simulink library "fmCopterAltHoldIndi_lib"  (R2018b)
settings: Solver=VariableStepAuto  StartTime=0.0  StopTime=10.0  RelTol=1e-3
undefined symbols (not defined in the file or in its folder): fm_alt_hold
libraries: filters_lib x5, indi_lib x1, cntrlAttiRedIndi_lib x1, cntrlAltIndi_lib x1
settings Model: Creator=Ybeyer  LastModifiedBy=yannic
settings SFSimCC: SimUseLocalCustomCode=off
settings RTWCC: RTWUseLocalCustomCode=off
settings CodeAppCC: StateflowObjectComments=on

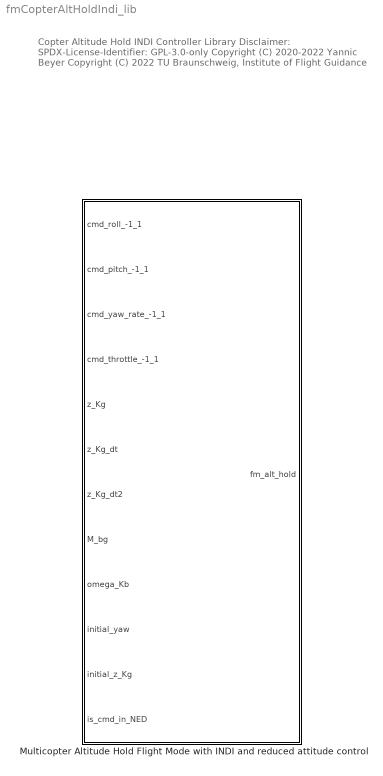
== system fmCopterAltHoldIndi_lib ==
  note: Copter Altitude Hold INDI Controller Library
      |
      | Disclaimer:
      | SPDX-License-Identifier: GPL-3.0-only
      |
      | Copyright (C) 2020-2022 Yannic Beyer
      | Copyright (C) 2022 TU Braunschweig, Institute of Flight Guidance
  Multicopter Altitude Hold Flight Mode with INDI and reduced attitude control : Subsystem  mask{fm=fm_alt_hold}
      mask prompts: fm "Multicopter Altitude Hold Flight Mode (INDI) struct, see fmCopterAltHoldIndi_params_default"
      mask DialogControl DescGroupVar Prompt: Multicopter Attitude Flight Mode with INDI and reduced attitude control
      mask DialogControl DescTextVar Prompt: Controller is basically implemented according to [1]
      mask DialogControl Control2 Prompt: [1] Sun, S., Baert, M., Van Schijndel, B. S., & De Visser, C. (2020, May). Upset Recovery Control for Quadrotors Subjected to a Complete Rotor Failure from Large Initial Disturbances. In 2020 IEEE International Conference on Robotics and Automation (ICRA) (pp. 4273-4279). IEEE.

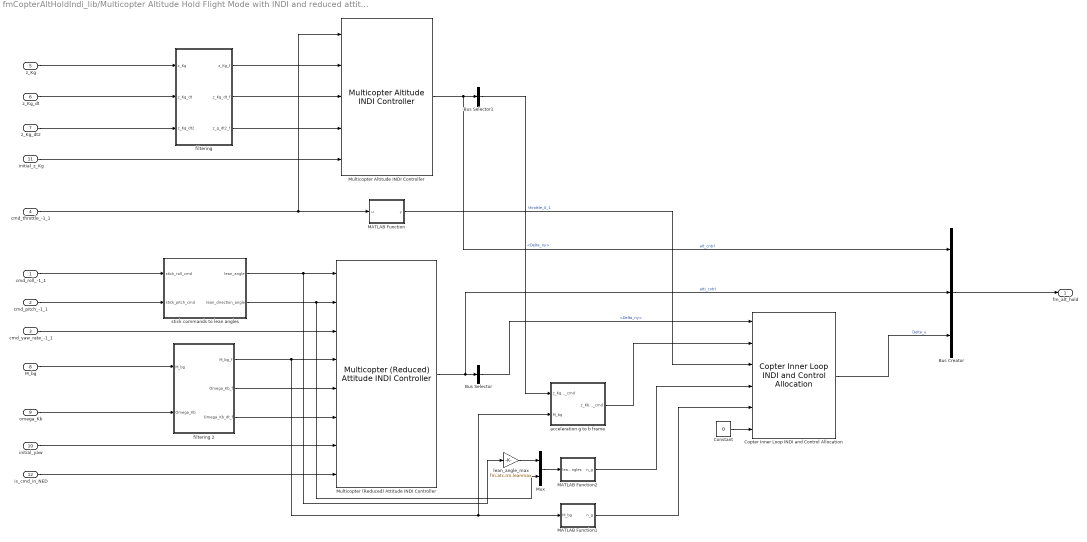
== system fmCopterAltHoldIndi_lib/Multicopter Altitude Hold Flight Mode with INDI and reduced attitude control ==
  cmd_roll_-1_1 : Inport  SampleTime=fm.ts
  cmd_pitch_-1_1 : Inport  Port=2  SampleTime=fm.ts
  cmd_yaw_rate_-1_1 : Inport  Port=3  SampleTime=fm.ts
  cmd_throttle_-1_1 : Inport  Port=4  SampleTime=fm.ts
  z_Kg : Inport  Port=5  SampleTime=fm.ts
  z_Kg_dt : Inport  Port=6  SampleTime=fm.ts
  z_Kg_dt2 : Inport  Port=7  SampleTime=fm.ts
  M_bg : Inport  Port=8  SampleTime=fm.ts
  omega_Kb : Inport  Port=9  SampleTime=fm.ts
  initial_yaw : Inport  Port=10  SampleTime=fm.ts
  initial_z_Kg : Inport  Port=11  SampleTime=fm.ts
  is_cmd_in_NED : Inport  Port=12  SampleTime=fm.ts
  Bus Creator : BusCreator  Inputs=3
  Bus Selector : BusSelector  OutputSignals=pseudo_control.Delta_ny
  Bus Selector1 : BusSelector  OutputSignals=pseudo_control.Delta_ny
  Constant : Constant  Value=0
  Copter Inner Loop INDI and Control Allocation : indi_lib/Copter Inner Loop INDI and Control Allocation  cep=fm.cep  ceb=fm.ceb  ca=fm.ca  mtc=fm.mtc  sflt=fm.sflt  ts=fm.ts
      settings: SourceProductName=LADAC
  MATLAB Function : MATLAB Function  TreatAsAtomicUnit=on
  MATLAB Function1 : MATLAB Function  TreatAsAtomicUnit=on
  MATLAB Function2 : MATLAB Function  TreatAsAtomicUnit=on
  Multicopter (Reduced) Attitude INDI Controller : cntrlAttiRedIndi_lib/Multicopter (Reduced) Attitude INDI Controller  atc=fm.atc  T=fm.mtc + 2./fm.sflt.omega
      settings: SourceProductName=LADAC
  Multicopter Altitude INDI Controller : cntrlAltIndi_lib/Multicopter Altitude INDI Controller  psc=fm.psc
      settings: SourceProductName=LADAC
  Mux : Mux  Inputs=2
  acceleration g to b frame : Subsystem
  filtering : Subsystem
  filtering 2 : Subsystem
  lean_angle_max : Gain  Gain=fm.atc.rm.leanmax
  stick commands to lean angles : MATLAB Function  TreatAsAtomicUnit=on
  fm_alt_hold : Outport  SampleTime=fm.ts
  wires:
  is_cmd_in_NED/1 -> Multicopter (Reduced) Attitude INDI Controller/8
  Multicopter Altitude INDI Controller/1 -> Bus Creator/1, Bus Selector1/1  "alt_cntrl"
  cmd_yaw_rate_-1_1/1 -> Multicopter (Reduced) Attitude INDI Controller/3
  stick commands to lean angles/2(lean_direction_angle) -> Mux/2, Multicopter (Reduced) Attitude INDI Controller/2
  Bus Selector1/1 -> acceleration g to b frame/1(z_Kg_dt2_cmd)  "<Delta_ny>"
  MATLAB Function/1(y) -> Copter Inner Loop INDI and Control Allocation/3  "throttle_0_1"
  cmd_throttle_-1_1/1 -> MATLAB Function/1(u), Multicopter Altitude INDI Controller/1
  Multicopter (Reduced) Attitude INDI Controller/1 -> Bus Creator/2, Bus Selector/1  "atti_cntrl"
  initial_yaw/1 -> Multicopter (Reduced) Attitude INDI Controller/7
  stick commands to lean angles/1(lean_angle) -> lean_angle_max/1, Multicopter (Reduced) Attitude INDI Controller/1
  Bus Selector/1 -> Copter Inner Loop INDI and Control Allocation/1  "<Delta_ny>"
  filtering 2/3(Omega_Kb_dt_f) -> Multicopter (Reduced) Attitude INDI Controller/6
  filtering 2/2(Omega_Kb_f) -> Multicopter (Reduced) Attitude INDI Controller/5
  filtering/1(z_Kg_f) -> Multicopter Altitude INDI Controller/2
  filtering/2(z_Kg_dt_f) -> Multicopter Altitude INDI Controller/3
  filtering/3(z_g_dt2_f) -> Multicopter Altitude INDI Controller/4
  initial_z_Kg/1 -> Multicopter Altitude INDI Controller/5
  Bus Creator/1 -> fm_alt_hold/1
  cmd_roll_-1_1/1 -> stick commands to lean angles/1(stick_roll_cmd)
  cmd_pitch_-1_1/1 -> stick commands to lean angles/2(stick_pitch_cmd)
  filtering 2/1(M_bg_f) -> Multicopter (Reduced) Attitude INDI Controller/4, acceleration g to b frame/2(M_bg), MATLAB Function1/1(M_bg)
  acceleration g to b frame/1(z_Kb_dt2_cmd) -> Copter Inner Loop INDI and Control Allocation/2
  Copter Inner Loop INDI and Control Allocation/1 -> Bus Creator/3  "Delta_u"
  z_Kg/1 -> filtering/1(z_Kg)
  z_Kg_dt/1 -> filtering/2(z_Kg_dt)
  z_Kg_dt2/1 -> filtering/3(z_Kg_dt2)
  M_bg/1 -> filtering 2/1(M_bg)
  omega_Kb/1 -> filtering 2/2(Omega_Kb)
  MATLAB Function1/1(n_g) -> Copter Inner Loop INDI and Control Allocation/5
  MATLAB Function2/1(n_g) -> Copter Inner Loop INDI and Control Allocation/4
  lean_angle_max/1 -> Mux/1
  Mux/1 -> MATLAB Function2/1(leanAngles)
  Constant/1 -> Copter Inner Loop INDI and Control Allocation/6

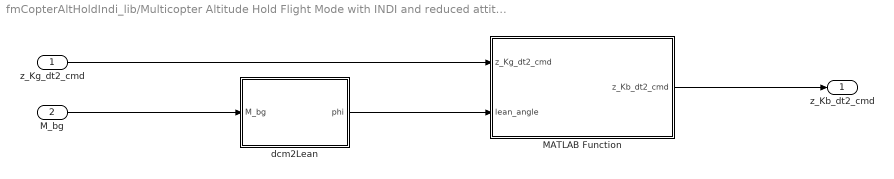
== system fmCopterAltHoldIndi_lib/Multicopter Altitude Hold Flight Mode with INDI and reduced attitude control/acceleration g to b frame ==
  z_Kg_dt2_cmd : Inport
  M_bg : Inport  Port=2
  MATLAB Function : MATLAB Function  TreatAsAtomicUnit=on
  dcm2Lean : MATLAB Function  TreatAsAtomicUnit=on
  z_Kb_dt2_cmd : Outport
  wires:
  z_Kg_dt2_cmd/1 -> MATLAB Function/1(z_Kg_dt2_cmd)
  MATLAB Function/1(z_Kb_dt2_cmd) -> z_Kb_dt2_cmd/1
  M_bg/1 -> dcm2Lean/1(M_bg)
  dcm2Lean/1(phi) -> MATLAB Function/2(lean_angle)

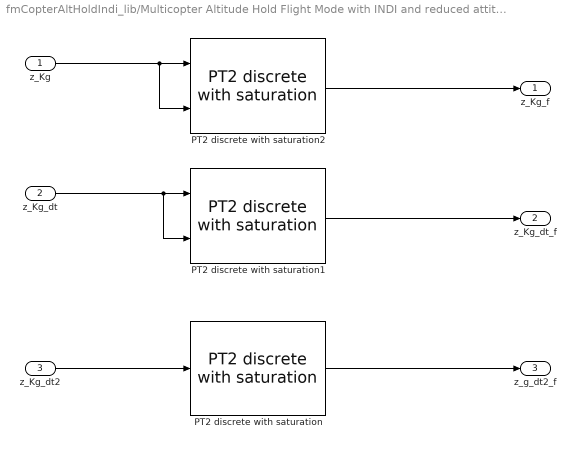
== system fmCopterAltHoldIndi_lib/Multicopter Altitude Hold Flight Mode with INDI and reduced attitude control/filtering ==
  z_Kg : Inport
  z_Kg_dt : Inport  Port=2
  z_Kg_dt2 : Inport  Port=3
  PT2 discrete with saturation : filters_lib/PT2 discrete with saturation  param_src=internal  omega=fm.sflt.omega  d=fm.sflt.D  x_dt2_max=inf  x_dt2_min=-inf  x_dt_max=inf  x_dt_min=-inf  x_max=inf  x_min=-inf  y_0_src=internal  x_init=0  y_dt_0_src=internal  x_dt_init=0  is_y_dt_checked=off  is_y_dt2_checked=off
      settings: SourceProductName=LADAC
  PT2 discrete with saturation1 : filters_lib/PT2 discrete with saturation  param_src=internal  omega=fm.sflt.omega  d=fm.sflt.D  x_dt2_max=inf  x_dt2_min=-inf  x_dt_max=inf  x_dt_min=-inf  x_max=inf  x_min=-inf  y_0_src=external  x_init=0  y_dt_0_src=internal  x_dt_init=0  is_y_dt_checked=off  is_y_dt2_checked=off
      settings: SourceProductName=LADAC
  PT2 discrete with saturation2 : filters_lib/PT2 discrete with saturation  param_src=internal  omega=fm.sflt.omega  d=fm.sflt.D  x_dt2_max=inf  x_dt2_min=-inf  x_dt_max=inf  x_dt_min=-inf  x_max=inf  x_min=-inf  y_0_src=external  x_init=0  y_dt_0_src=internal  x_dt_init=0  is_y_dt_checked=off  is_y_dt2_checked=off
      settings: SourceProductName=LADAC
  z_Kg_f : Outport
  z_Kg_dt_f : Outport  Port=2
  z_g_dt2_f : Outport  Port=3
  wires:
  PT2 discrete with saturation/1 -> z_g_dt2_f/1
  z_Kg_dt2/1 -> PT2 discrete with saturation/1
  PT2 discrete with saturation1/1 -> z_Kg_dt_f/1
  z_Kg_dt/1 -> PT2 discrete with saturation1/2, PT2 discrete with saturation1/1
  PT2 discrete with saturation2/1 -> z_Kg_f/1
  z_Kg/1 -> PT2 discrete with saturation2/1, PT2 discrete with saturation2/2

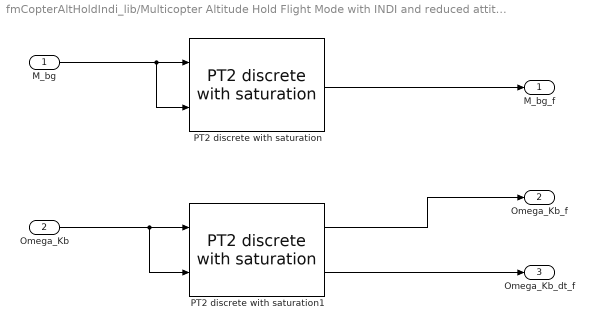
== system fmCopterAltHoldIndi_lib/Multicopter Altitude Hold Flight Mode with INDI and reduced attitude control/filtering 2 ==
  M_bg : Inport
  Omega_Kb : Inport  Port=2
  PT2 discrete with saturation : filters_lib/PT2 discrete with saturation  param_src=internal  omega=fm.sflt.omega  d=fm.sflt.D  x_dt2_max=inf  x_dt2_min=-inf  x_dt_max=inf  x_dt_min=-inf  x_max=inf  x_min=-inf  y_0_src=external  x_init=0  y_dt_0_src=internal  x_dt_init=0  is_y_dt_checked=off  is_y_dt2_checked=off
      settings: SourceProductName=LADAC
  PT2 discrete with saturation1 : filters_lib/PT2 discrete with saturation  param_src=internal  omega=fm.sflt.omega  d=fm.sflt.D  x_dt2_max=inf  x_dt2_min=-inf  x_dt_max=inf  x_dt_min=-inf  x_max=inf  x_min=-inf  y_0_src=external  x_init=0  y_dt_0_src=internal  x_dt_init=0  is_y_dt_checked=on  is_y_dt2_checked=off
      settings: SourceProductName=LADAC
  M_bg_f : Outport
  Omega_Kb_f : Outport  Port=2
  Omega_Kb_dt_f : Outport  Port=3
  wires:
  PT2 discrete with saturation1/2 -> Omega_Kb_dt_f/1
  Omega_Kb/1 -> PT2 discrete with saturation1/2, PT2 discrete with saturation1/1
  PT2 discrete with saturation1/1 -> Omega_Kb_f/1
  M_bg/1 -> PT2 discrete with saturation/2, PT2 discrete with saturation/1
  PT2 discrete with saturation/1 -> M_bg_f/1

== matlab function fmCopterAltHoldIndi_lib/Multicopter Altitude Hold Flight Mode with INDI and reduced attitude control/MATLAB Function1 ==
  data: M_bg input; n_g output
function n_g = dcm2LeanVector( M_bg )
n_g = dcm2LeanVector( M_bg );
end

== matlab function fmCopterAltHoldIndi_lib/Multicopter Altitude Hold Flight Mode with INDI and reduced attitude control/MATLAB Function ==
  data: u input; y output
function y = fcn(u)
y = 0.5*u+0.5;

== matlab function fmCopterAltHoldIndi_lib/Multicopter Altitude Hold Flight Mode with INDI and reduced attitude control/stick commands to lean angles ==
  data: stick_roll_cmd input; lean_angle output; stick_pitch_cmd input; lean_direction_angle output
function [lean_angle,lean_direction_angle] = fcn(stick_roll_cmd,stick_pitch_cmd)

lean_direction_angle = atan2(stick_roll_cmd,-stick_pitch_cmd);
lean_angle = sqrt( stick_roll_cmd^2 + stick_pitch_cmd^2 );

end

== matlab function fmCopterAltHoldIndi_lib/Multicopter Altitude Hold Flight Mode with INDI and reduced attitude control/acceleration g to b frame/MATLAB Function ==
  data: z_Kg_dt2_cmd input; z_Kb_dt2_cmd output; lean_angle input
function z_Kb_dt2_cmd = fcn(z_Kg_dt2_cmd,lean_angle)

% compensate lean angle
cos_lean = cos(lean_angle);
if cos_lean > 0.1
    z_Kb_dt2_cmd = z_Kg_dt2_cmd / cos_lean;
else
    z_Kb_dt2_cmd = z_Kg_dt2_cmd;
end

end

== matlab function fmCopterAltHoldIndi_lib/Multicopter Altitude Hold Flight Mode with INDI and reduced attitude control/acceleration g to b frame/dcm2Lean ==
  data: M_bg input; phi output
function phi= dcm2Lean( M_bg )
[phi,~] = dcm2Lean( M_bg );
end

== matlab function fmCopterAltHoldIndi_lib/Multicopter Altitude Hold Flight Mode with INDI and reduced attitude control/MATLAB Function2 ==
  data: leanAngles input; n_g output
function n_g = fcn( leanAngles )
n_g = leanAngles2leanVector( leanAngles );
end
